simulink model "sfir_half"  (R2026a)
settings: Solver=FixedStepDiscrete  StopTime=2000
Description:
  | Symmetric FIR Filter
  | This example shows how to use HDL Coder(TM) to check, generate,
  | and verify HDL for a fixed-point symmetric FIR filter.
settings Model: Creator=The MathWorks, Inc.  LastModifiedBy=The MathWorks, Inc.
settings DataIOCC: SignalLoggingName=logsOut
settings OptimizationCC: BooleanDataType=off  ConditionallyExecuteInputs=off  InlineInvariantSignals=on  InitFltsAndDblsToZero=on  BufferReusableBoundary=off
settings DebuggingCC: AlgebraicLoopMsg=error  SaveWithParameterizedLinksMsg=none  UnderspecifiedInitializationDetection=Classic  CheckExecutionContextPreStartOutputMsg=on  SignalResolutionControl=TryResolveAllWithWarning  MultiTaskDSMMsg=warning  MultiTaskCondExecSysMsg=none  SingleTaskRateTransMsg=error  IntegerOverflowMsg=none  ParameterPrecisionLossMsg=none  BusObjectLabelMismatch=none  IntegerSaturationMsg=none
settings HardwareCC: ProdHWDeviceType=ASIC/FPGA  TargetUnknown=on  ProdEqTarget=off
settings GRTTargetCC: TargetFcnLib=ansi_tfl_tmw.mat  CombineOutputUpdateFcns=off  GRTInterface=on

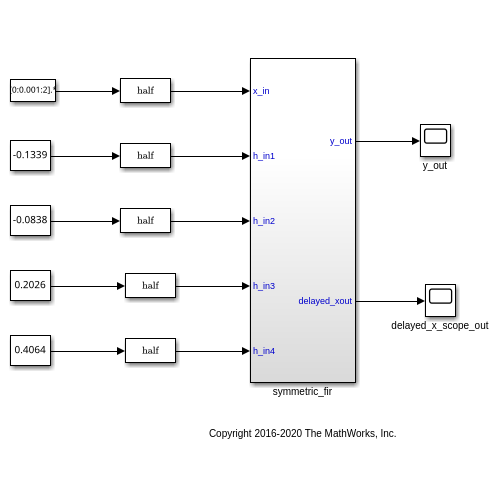
[thumbnail: Simulink's stored preview of the top-level diagram]
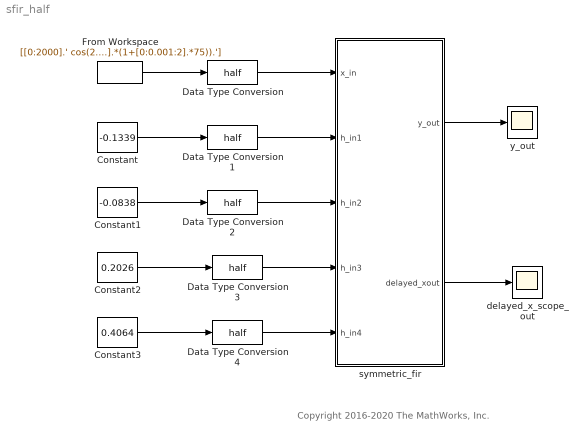
== system sfir_half ==
  note: Copyright 2016-2020 The MathWorks, Inc.
  Constant : Constant  Value=-0.1339  OutDataTypeStr=fixdt(1,16,10)  SampleTime=1
  Constant1 : Constant  Value=-0.0838  OutDataTypeStr=fixdt(1,16,10)  SampleTime=1
  Constant2 : Constant  Value=0.2026  OutDataTypeStr=fixdt(1,16,10)  SampleTime=1
  Constant3 : Constant  Value=0.4064  OutDataTypeStr=fixdt(1,16,10)  SampleTime=1
  Data Type Conversion{,1..4} (5 alike) : DataTypeConversion  OutDataTypeStr=half  SaturateOnIntegerOverflow=off  RndMeth=Floor
  From Workspace : FromWorkspace  VariableName=[[0:2000].' cos(2.*pi.*[0:0.001:2].*(1+[0:0.001:2].*75)).']  SampleTime=1  OutputAfterFinalValue=Setting to zero
  delayed_x_scope_out : Scope
  symmetric_fir : Subsystem
  y_out : Scope
      settings: ActiveDisplayYMinimum=-1.51817  ActiveDisplayYMaximum=1.51898
  wires:
  Constant1/1 -> Data Type Conversion2/1
  Constant3/1 -> Data Type Conversion4/1
  Constant2/1 -> Data Type Conversion3/1
  symmetric_fir/1(y_out) -> y_out/1
  symmetric_fir/2(delayed_xout) -> delayed_x_scope_out/1
  Constant/1 -> Data Type Conversion1/1
  From Workspace/1 -> Data Type Conversion/1
  Data Type Conversion/1 -> symmetric_fir/1(x_in)
  Data Type Conversion1/1 -> symmetric_fir/2(h_in1)
  Data Type Conversion2/1 -> symmetric_fir/3(h_in2)
  Data Type Conversion3/1 -> symmetric_fir/4(h_in3)
  Data Type Conversion4/1 -> symmetric_fir/5(h_in4)

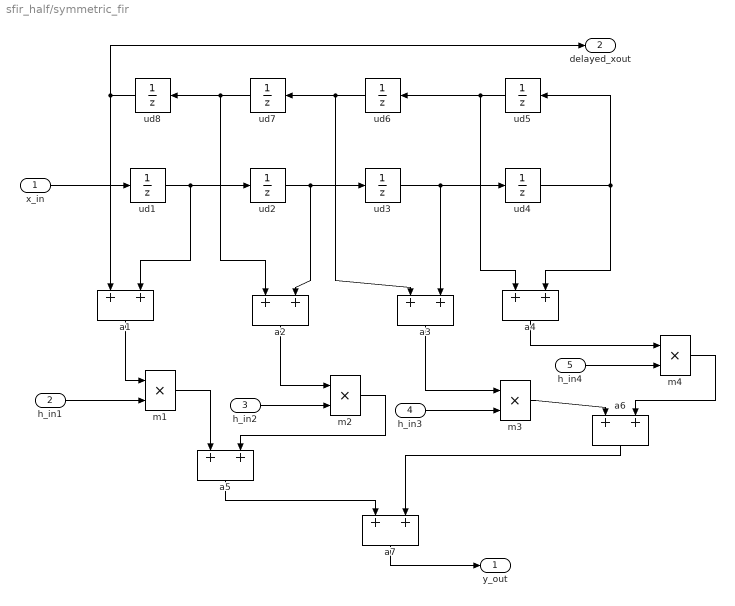
== system sfir_half/symmetric_fir ==
  x_in : Inport
  h_in1 : Inport  Port=2
  h_in2 : Inport  Port=3
  h_in3 : Inport  Port=4
  h_in4 : Inport  Port=5
  a{1..7} (7 alike) : Sum  OutDataTypeStr=half
  m{1..4} (4 alike) : Product  OutDataTypeStr=half  RndMeth=Zero
  ud{1..8} (8 alike) : UnitDelay  SampleTime=-1
  y_out : Outport  VectorParamsAs1DForOutWhenUnconnected=off
  delayed_xout : Outport  Port=2  VectorParamsAs1DForOutWhenUnconnected=off
  wires:
  a4/1 -> m4/1
  ud7/1 -> a2/1, ud8/1
  ud6/1 -> a3/1, ud7/1
  ud5/1 -> a4/1, ud6/1
  ud2/1 -> a2/2, ud3/1
  ud4/1 -> a4/2, ud5/1
  ud8/1 -> a1/1, delayed_xout/1
  a3/1 -> m3/1
  ud3/1 -> a3/2, ud4/1
  a2/1 -> m2/1
  a1/1 -> m1/1
  m1/1 -> a5/1
  m2/1 -> a5/2
  m3/1 -> a6/1
  m4/1 -> a6/2
  a5/1 -> a7/1
  a6/1 -> a7/2
  a7/1 -> y_out/1
  h_in1/1 -> m1/2
  h_in2/1 -> m2/2
  h_in3/1 -> m3/2
  h_in4/1 -> m4/2
  ud1/1 -> a1/2, ud2/1
  x_in/1 -> ud1/1
